simulink model "ACC_FFNN_trainlm_10_10_10_Nor_Sat_Feb_15_RepFast"  (R2021a)
settings: Solver=FixedStepAuto  StartTime=0.0  StopTime=T  RelTol=1e-3
InitFcn:
  | seed = randi(10000);
StartFcn:
  | seed = randi(10000);
undefined symbols (not defined in the file): amax_ego, amin_ego, patch_sig, safe_patch_sig, sw, t_gap, Ts, v0_ego, v0_lead, v_set, x0_ego, x0_lead, x_gain, x_offset, y_gain, y_offset
libraries: neural x35, simulink x3
(part 1 of 2)
settings Model: SimulationMode=accelerator  Creator=The MathWorks, Inc.  LastModifiedBy=deyun
settings SolverCC: AlgebraicLoopSolver=TrustRegion
settings DataIOCC: ReturnWorkspaceOutputs=off
settings DebuggingCC: ArithmeticOperatorsInVariantConditions=warning
settings SFSimCC: SimUseLocalCustomCode=off  CustomCodeUndefinedFunction=UseInterfaceOnly
settings RTWCC: RTWUseLocalCustomCode=off
settings CodeAppCC: StateflowObjectComments=on
settings ConfigComp: CovBoundaryAbsTol=1.0e-5

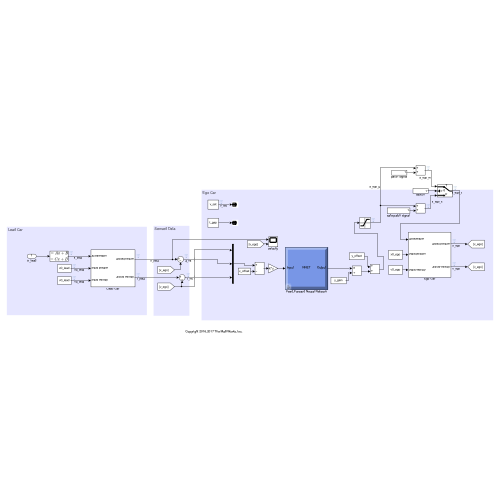
[thumbnail: Simulink's stored preview of the top-level diagram]
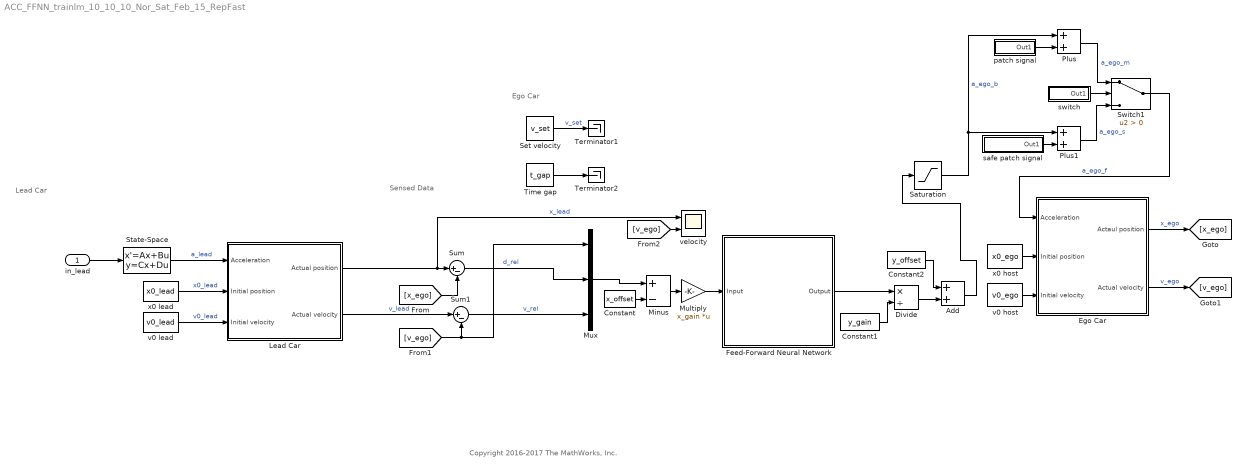
== system ACC_FFNN_trainlm_10_10_10_Nor_Sat_Feb_15_RepFast ==
  note: Sensed Data
  note: Lead Car
  note: Ego Car
  note: Copyright 2016-2017 The MathWorks, Inc.
  in_lead : Inport
  Add : Sum
  Constant : Constant  Value=x_offset
  Constant1 : Constant  Value=y_gain
  Constant2 : Constant  Value=y_offset
  Divide : Product  Inputs=*/
  Ego Car : Subsystem
  Feed-Forward Neural Network : Subsystem
      mask help: Feed-Forward Neural Network
      mask Display: e = 0.06;c1 = [120 150 230]/255;c2 = ([120 150 230]+0)/383;c3 = ([120 150 230]+128)/383;patch([0 1 1 0],[0 0 1 1],c1);patch([0 1 1 1-e 1-e 0+e],[0 0 1 1-e 0+e 0+e],c2);patch([0 0 1 1-e 0+e 0+e],[0 1 1 1-e 1-e 0+e],c3);plot([0 1 1 0 0],[0 0 1 1 0]);fprintf('NNET');port_label('input',1,' Input');port_label('output',1,'Output ');
  Lead Car : Subsystem
  Minus : Sum  Inputs=+-
  Multiply : Gain  Gain=x_gain  Multiplication=Matrix(K*u)
  Mux : Mux  Inputs=3
  Plus : Sum
  Plus1 : Sum
  Saturation : Saturate  UpperLimit=amax_ego  LowerLimit=amin_ego
  Set velocity : Constant  Value=v_set  SampleTime=Ts
  State-Space : StateSpace  A=-10  B=10  D=0  InitialCondition=0
  Sum : Sum  Inputs=|+-
  Sum1 : Sum  Inputs=|+-
  Switch1 : Switch  Criteria=u2 > Threshold
  Terminator1 : Terminator
  Terminator2 : Terminator
  Time gap : Constant  Value=t_gap  SampleTime=Ts
  patch signal : Subsystem
  safe patch signal : Subsystem
  switch : Subsystem
  v0 host : Constant  Value=v0_ego  SampleTime=Ts
  v0 lead : Constant  Value=v0_lead  SampleTime=Ts
  velocity : Scope  NumInputPorts=2
  x0 host : Constant  Value=x0_ego  SampleTime=Ts
  x0 lead : Constant  Value=x0_lead  SampleTime=Ts
  wires:
  x0 lead/1 -> Lead Car/2(Initial position)  "x0_lead"
  v0 lead/1 -> Lead Car/3(Initial velocity)  "v0_lead"
  x0 host/1 -> Ego Car/2(Initial position)
  v0 host/1 -> Ego Car/3(Initial velocity)
  Feed-Forward Neural Network/1(Output) -> Divide/1
  Lead Car/1(Actual position) -> velocity/1, Sum/1  "x_lead"
  Sum1/1 -> Mux/3  "v_rel"
  State-Space/1 -> Lead Car/1(Acceleration)  "a_lead"
  Lead Car/2(Actual velocity) -> Sum1/1  "v_lead"
  in_lead/1 -> State-Space/1
  Mux/1 -> Minus/1
  Add/1 -> Saturation/1
  Multiply/1 -> Feed-Forward Neural Network/1(Input)
  Set velocity/1 -> Terminator1/1  "v_set"
  Time gap/1 -> Terminator2/1
  Constant/1 -> Minus/2
  Minus/1 -> Multiply/1
  Constant1/1 -> Divide/2
  Divide/1 -> Add/2
  Constant2/1 -> Add/1
  Ego Car/1(Actaul position) -> [x_ego]  "x_ego"
  [x_ego] -> Sum/2
  Ego Car/2(Actual velocity) -> [v_ego]  "v_ego"
  [v_ego] -> Mux/1, Sum1/2
  [v_ego] -> velocity/2
  Sum/1 -> Mux/2  "d_rel"
  Saturation/1 -> Plus/1, Plus1/1  "a_ego_b"
  Plus1/1 -> Switch1/3  "a_ego_s"
  Switch1/1 -> Ego Car/1(Acceleration)  "a_ego_f"
  Plus/1 -> Switch1/1  "a_ego_m"
  patch signal/1(Out1) -> Plus/2
  safe patch signal/1(Out1) -> Plus1/2
  switch/1(Out1) -> Switch1/2

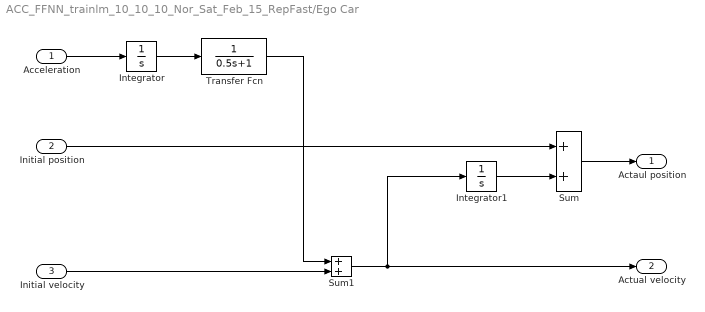
== system ACC_FFNN_trainlm_10_10_10_Nor_Sat_Feb_15_RepFast/Ego Car ==
  Acceleration : Inport
  Initial position : Inport  Port=2
  Initial velocity : Inport  Port=3
  Integrator : Integrator
  Integrator1 : Integrator
  Sum : Sum
  Sum1 : Sum
  Transfer Fcn : TransferFcn  Denominator=[0.5 1]
  Actaul position : Outport  VectorParamsAs1DForOutWhenUnconnected=off
  Actual velocity : Outport  Port=2  VectorParamsAs1DForOutWhenUnconnected=off
  wires:
  Sum1/1 -> Integrator1/1, Actual velocity/1
  Initial velocity/1 -> Sum1/2
  Sum/1 -> Actaul position/1
  Transfer Fcn/1 -> Sum1/1
  Integrator/1 -> Transfer Fcn/1
  Acceleration/1 -> Integrator/1
  Initial position/1 -> Sum/1
  Integrator1/1 -> Sum/2

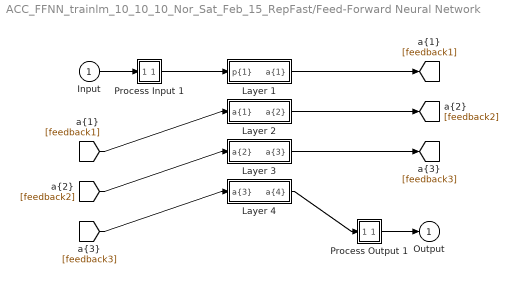
== system ACC_FFNN_trainlm_10_10_10_Nor_Sat_Feb_15_RepFast/Feed-Forward Neural Network ==
  Input : Inport  PortDimensions=3
      mask Display: e = 0.06;c1 = [120 230 180]/255;c2 = ([120 230 180]+0)/(256+128);c3 = ([120 230 180]+128)/(256+128);patch([0 1 1 0],[0 0 1 1],c1);patch([0 1 1 1-e 1-e 0+e],[0 0 1 1-e 0+e 0+e],c2);patch([0 0 1 1-e 0+e 0+e],[0 1 1 1-e 1-e 0+e],c3);plot([0 1 1 0 0],[0 0 1 1 0]);
  Layer 1 : Subsystem
      mask Display: e = 0.06;c1 = [120 150 230]/255;c2 = ([120 150 230]+0)/383;c3 = ([120 150 230]+128)/383;patch([0 1 1 0],[0 0 1 1],c1);patch([0 1 1 1-e 1-e 0+e],[0 0 1 1-e 0+e 0+e],c2);patch([0 0 1 1-e 0+e 0+e],[0 1 1 1-e 1-e 0+e],c3);plot([0 1 1 0 0],[0 0 1 1 0]);
  Layer 2 : Subsystem
      mask Display: e = 0.06;c1 = [120 150 230]/255;c2 = ([120 150 230]+0)/383;c3 = ([120 150 230]+128)/383;patch([0 1 1 0],[0 0 1 1],c1);patch([0 1 1 1-e 1-e 0+e],[0 0 1 1-e 0+e 0+e],c2);patch([0 0 1 1-e 0+e 0+e],[0 1 1 1-e 1-e 0+e],c3);plot([0 1 1 0 0],[0 0 1 1 0]);
  Layer 3 : Subsystem
      mask Display: e = 0.06;c1 = [120 150 230]/255;c2 = ([120 150 230]+0)/383;c3 = ([120 150 230]+128)/383;patch([0 1 1 0],[0 0 1 1],c1);patch([0 1 1 1-e 1-e 0+e],[0 0 1 1-e 0+e 0+e],c2);patch([0 0 1 1-e 0+e 0+e],[0 1 1 1-e 1-e 0+e],c3);plot([0 1 1 0 0],[0 0 1 1 0]);
  Layer 4 : Subsystem
      mask Display: e = 0.06;c1 = [120 150 230]/255;c2 = ([120 150 230]+0)/383;c3 = ([120 150 230]+128)/383;patch([0 1 1 0],[0 0 1 1],c1);patch([0 1 1 1-e 1-e 0+e],[0 0 1 1-e 0+e 0+e],c2);patch([0 0 1 1-e 0+e 0+e],[0 1 1 1-e 1-e 0+e],c3);plot([0 1 1 0 0],[0 0 1 1 0]);
  Process Input 1 : Subsystem
      mask Display: e = 0.06;c1 = [120 150 230]/255;c2 = ([120 150 230]+0)/383;c3 = ([120 150 230]+128)/383;patch([0 1 1 0],[0 0 1 1],c1);patch([0 1 1 1-e 1-e 0+e],[0 0 1 1-e 0+e 0+e],c2);patch([0 0 1 1-e 0+e 0+e],[0 1 1 1-e 1-e 0+e],c3);plot([0 1 1 0 0],[0 0 1 1 0]);
  Process Output 1 : Subsystem
      mask Display: e = 0.06;c1 = [120 150 230]/255;c2 = ([120 150 230]+0)/383;c3 = ([120 150 230]+128)/383;patch([0 1 1 0],[0 0 1 1],c1);patch([0 1 1 1-e 1-e 0+e],[0 0 1 1-e 0+e 0+e],c2);patch([0 0 1 1-e 0+e 0+e],[0 1 1 1-e 1-e 0+e],c3);plot([0 1 1 0 0],[0 0 1 1 0]);
  Output : Outport  InitialOutput=0
      mask Display: e = 0.06;c1 = [120 230 180]/255;c2 = ([120 230 180]+0)/(256+128);c3 = ([120 230 180]+128)/(256+128);patch([0 1 1 0],[0 0 1 1],c1);patch([0 1 1 1-e 1-e 0+e],[0 0 1 1-e 0+e 0+e],c2);patch([0 0 1 1-e 0+e 0+e],[0 1 1 1-e 1-e 0+e],c3);plot([0 1 1 0 0],[0 0 1 1 0]);
  wires:
  Input/1 -> Process Input 1/1(x)
  Process Output 1/1(y) -> Output/1
  Process Input 1/1(p) -> Layer 1/1("p{1}")
  Layer 1/1("a{1}") -> [feedback1]
  [feedback1] -> Layer 2/1("a{1} ")
  Layer 2/1("a{2}") -> [feedback2]
  [feedback2] -> Layer 3/1("a{2} ")
  Layer 3/1("a{3}") -> [feedback3]
  [feedback3] -> Layer 4/1("a{3} ")
  Layer 4/1("a{4}") -> Process Output 1/1(a)

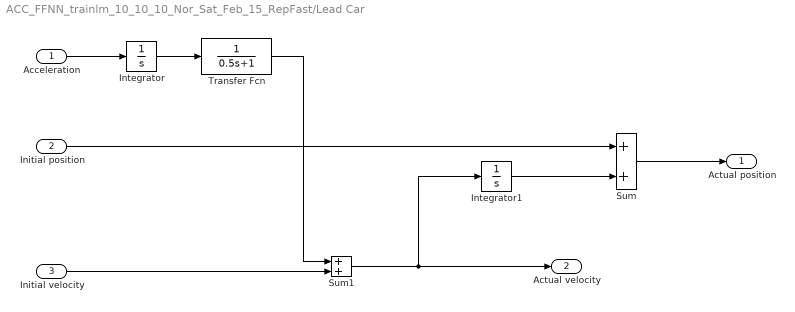
== system ACC_FFNN_trainlm_10_10_10_Nor_Sat_Feb_15_RepFast/Lead Car ==
  Acceleration : Inport
  Initial position : Inport  Port=2
  Initial velocity : Inport  Port=3
  Integrator : Integrator
  Integrator1 : Integrator
  Sum : Sum
  Sum1 : Sum
  Transfer Fcn : TransferFcn  Denominator=[0.5 1]
  Actual position : Outport  VectorParamsAs1DForOutWhenUnconnected=off
  Actual velocity : Outport  Port=2  VectorParamsAs1DForOutWhenUnconnected=off
  wires:
  Transfer Fcn/1 -> Sum1/1
  Initial velocity/1 -> Sum1/2
  Sum/1 -> Actual position/1
  Integrator/1 -> Transfer Fcn/1
  Sum1/1 -> Integrator1/1, Actual velocity/1
  Acceleration/1 -> Integrator/1
  Initial position/1 -> Sum/1
  Integrator1/1 -> Sum/2

== system ACC_FFNN_trainlm_10_10_10_Nor_Sat_Feb_15_RepFast/patch signal ==
  Sample index : simulink/Sources/Counter Limited  uplimit=numel(patch_sig)-1  tsamp=Ts
  Sample value : LookupNDDirect  NumberOfTableDimensions=1  Table=patch_sig  DiagnosticForOutOfRangeInput=None
  Out1 : Outport
  wires:
  Sample index/1 -> Sample value/1
  Sample value/1 -> Out1/1

== system ACC_FFNN_trainlm_10_10_10_Nor_Sat_Feb_15_RepFast/safe patch signal ==
  Sample index : simulink/Sources/Counter Limited  uplimit=numel(safe_patch_sig)-1  tsamp=Ts
  Sample value : LookupNDDirect  NumberOfTableDimensions=1  Table=safe_patch_sig  DiagnosticForOutOfRangeInput=None
  Out1 : Outport
  wires:
  Sample index/1 -> Sample value/1
  Sample value/1 -> Out1/1

== system ACC_FFNN_trainlm_10_10_10_Nor_Sat_Feb_15_RepFast/switch ==
  Sample index : simulink/Sources/Counter Limited  uplimit=numel(sw)-1  tsamp=Ts
  Sample value : LookupNDDirect  NumberOfTableDimensions=1  Table=sw  DiagnosticForOutOfRangeInput=None
  Out1 : Outport
  wires:
  Sample index/1 -> Sample value/1
  Sample value/1 -> Out1/1

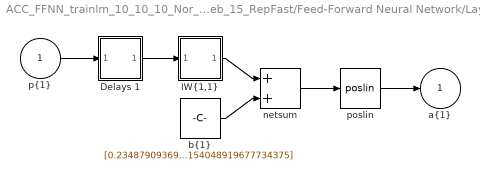
== system ACC_FFNN_trainlm_10_10_10_Nor_Sat_Feb_15_RepFast/Feed-Forward Neural Network/Layer 1 ==
  "p{1}" : Inport  PortDimensions=3
      mask Display: e = 0.06;c1 = [120 230 180]/255;c2 = ([120 230 180]+0)/(256+128);c3 = ([120 230 180]+128)/(256+128);patch([0 1 1 0],[0 0 1 1],c1);patch([0 1 1 1-e 1-e 0+e],[0 0 1 1-e 0+e 0+e],c2);patch([0 0 1 1-e 0+e 0+e],[0 1 1 1-e 1-e 0+e],c3);plot([0 1 1 0 0],[0 0 1 1 0]);
  Delays 1 : Subsystem
      mask Display: e = 0.06;c1 = [120 150 230]/255;c2 = ([120 150 230]+0)/383;c3 = ([120 150 230]+128)/383;patch([0 1 1 0],[0 0 1 1],c1);patch([0 1 1 1-e 1-e 0+e],[0 0 1 1-e 0+e 0+e],c2);patch([0 0 1 1-e 0+e 0+e],[0 1 1 1-e 1-e 0+e],c3);plot([0 1 1 0 0],[0 0 1 1 0]);disp('0');
  "IW{1,1}" : Subsystem
      mask Display: e = 0.06;c1 = [120 150 230]/255;c2 = ([120 150 230]+0)/383;c3 = ([120 150 230]+128)/383;patch([0 1 1 0],[0 0 1 1],c1);patch([0 1 1 1-e 1-e 0+e],[0 0 1 1-e 0+e 0+e],c2);patch([0 0 1 1-e 0+e 0+e],[0 1 1 1-e 1-e 0+e],c3);plot([0 1 1 0 0],[0 0 1 1 0]);disp('W');
  "b{1}" : Constant  Value=[0.2348790936912676652337239602275076322257518768310546875;-0.47557650443830912223575069219805300235748291015625;0.78952949301104913271132090812898240983486175537109375;0.27963461410623235980921208465588279068470001220703125;-0.65288334165578765233561853165156207978725433349609375;-0.6252719481796160660991290569654665887355804443359375;-0.285681783449709458810872320100315846502780914306640625;-0.362443396148235397191683659912087023258209228515625;-0.169633536236455551016177878409507684409618377685546875;0.07730292547507398859263361146076931618154048919677734375]
      mask Display: e = 0.06;c1 = [120 150 230]/255;c2 = ([120 150 230]+0)/383;c3 = ([120 150 230]+128)/383;patch([0 1 1 0],[0 0 1 1],c1);patch([0 1 1 1-e 1-e 0+e],[0 0 1 1-e 0+e 0+e],c2);patch([0 0 1 1-e 0+e 0+e],[0 1 1 1-e 1-e 0+e],c3);plot([0 1 1 0 0],[0 0 1 1 0]);disp('b');
  netsum : Sum  Inputs=2  InputSameDT=on  SaturateOnIntegerOverflow=on  OutDataTypeStr=Inherit: Same as first input
      mask Display: e = 0.06;c1 = [120 150 230]/255;c2 = ([120 150 230]+0)/383;c3 = ([120 150 230]+128)/383;patch([0 1 1 0],[0 0 1 1],c1);patch([0 1 1 1-e 1-e 0+e],[0 0 1 1-e 0+e 0+e],c2);patch([0 0 1 1-e 0+e 0+e],[0 1 1 1-e 1-e 0+e],c3);plot([0 1 1 0 0],[0 0 1 1 0]);disp('+');
  poslin : neural/Transfer Functions/poslin
  "a{1}" : Outport  InitialOutput=[0;0;0;0;0;0;0;0;0;0]
      mask Display: e = 0.06;c1 = [120 230 180]/255;c2 = ([120 230 180]+0)/(256+128);c3 = ([120 230 180]+128)/(256+128);patch([0 1 1 0],[0 0 1 1],c1);patch([0 1 1 1-e 1-e 0+e],[0 0 1 1-e 0+e 0+e],c2);patch([0 0 1 1-e 0+e 0+e],[0 1 1 1-e 1-e 0+e],c3);plot([0 1 1 0 0],[0 0 1 1 0]);
  wires:
  "p{1}"/1 -> Delays 1/1("p{1}")
  Delays 1/1("pd{1,1}") -> "IW{1,1}"/1("pd{1,1}")
  "IW{1,1}"/1("iz{1,1}") -> netsum/1
  "b{1}"/1 -> netsum/2
  netsum/1 -> poslin/1
  poslin/1 -> "a{1}"/1

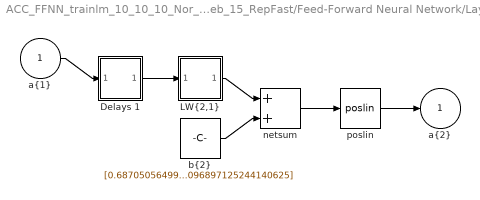
== system ACC_FFNN_trainlm_10_10_10_Nor_Sat_Feb_15_RepFast/Feed-Forward Neural Network/Layer 2 ==
  "a{1} " : Inport  PortDimensions=10
      mask Display: e = 0.06;c1 = [120 230 180]/255;c2 = ([120 230 180]+0)/(256+128);c3 = ([120 230 180]+128)/(256+128);patch([0 1 1 0],[0 0 1 1],c1);patch([0 1 1 1-e 1-e 0+e],[0 0 1 1-e 0+e 0+e],c2);patch([0 0 1 1-e 0+e 0+e],[0 1 1 1-e 1-e 0+e],c3);plot([0 1 1 0 0],[0 0 1 1 0]);
  Delays 1 : Subsystem
      mask Display: e = 0.06;c1 = [120 150 230]/255;c2 = ([120 150 230]+0)/383;c3 = ([120 150 230]+128)/383;patch([0 1 1 0],[0 0 1 1],c1);patch([0 1 1 1-e 1-e 0+e],[0 0 1 1-e 0+e 0+e],c2);patch([0 0 1 1-e 0+e 0+e],[0 1 1 1-e 1-e 0+e],c3);plot([0 1 1 0 0],[0 0 1 1 0]);disp('0');
  "LW{2,1}" : Subsystem
      mask Display: e = 0.06;c1 = [120 150 230]/255;c2 = ([120 150 230]+0)/383;c3 = ([120 150 230]+128)/383;patch([0 1 1 0],[0 0 1 1],c1);patch([0 1 1 1-e 1-e 0+e],[0 0 1 1-e 0+e 0+e],c2);patch([0 0 1 1-e 0+e 0+e],[0 1 1 1-e 1-e 0+e],c3);plot([0 1 1 0 0],[0 0 1 1 0]);disp('W');
  "b{2}" : Constant  Value=[0.68705056499902916744559888684307225048542022705078125;0.94653343063350003916411878890357911586761474609375;-0.94981534008346379938103609674726612865924835205078125;0.43723562506075897005075603374280035495758056640625;-0.46176114720288818915605588699690997600555419921875;-0.360550158804355092012627892472664825618267059326171875;-0.214341347450948627173517024857574142515659332275390625;1.1655184078745570719348734201048500835895538330078125;-0.1645117913666755971036081973579712212085723876953125;1.350983412230919444851906519033946096897125244140625]
      mask Display: e = 0.06;c1 = [120 150 230]/255;c2 = ([120 150 230]+0)/383;c3 = ([120 150 230]+128)/383;patch([0 1 1 0],[0 0 1 1],c1);patch([0 1 1 1-e 1-e 0+e],[0 0 1 1-e 0+e 0+e],c2);patch([0 0 1 1-e 0+e 0+e],[0 1 1 1-e 1-e 0+e],c3);plot([0 1 1 0 0],[0 0 1 1 0]);disp('b');
  netsum : Sum  Inputs=2  InputSameDT=on  SaturateOnIntegerOverflow=on  OutDataTypeStr=Inherit: Same as first input
      mask Display: e = 0.06;c1 = [120 150 230]/255;c2 = ([120 150 230]+0)/383;c3 = ([120 150 230]+128)/383;patch([0 1 1 0],[0 0 1 1],c1);patch([0 1 1 1-e 1-e 0+e],[0 0 1 1-e 0+e 0+e],c2);patch([0 0 1 1-e 0+e 0+e],[0 1 1 1-e 1-e 0+e],c3);plot([0 1 1 0 0],[0 0 1 1 0]);disp('+');
  poslin : neural/Transfer Functions/poslin
  "a{2}" : Outport  InitialOutput=[0;0;0;0;0;0;0;0;0;0]
      mask Display: e = 0.06;c1 = [120 230 180]/255;c2 = ([120 230 180]+0)/(256+128);c3 = ([120 230 180]+128)/(256+128);patch([0 1 1 0],[0 0 1 1],c1);patch([0 1 1 1-e 1-e 0+e],[0 0 1 1-e 0+e 0+e],c2);patch([0 0 1 1-e 0+e 0+e],[0 1 1 1-e 1-e 0+e],c3);plot([0 1 1 0 0],[0 0 1 1 0]);
  wires:
  "a{1} "/1 -> Delays 1/1("p{2}")
  Delays 1/1("pd{2,1}") -> "LW{2,1}"/1("ad{2,1}")
  "LW{2,1}"/1("lz{2,1}") -> netsum/1
  "b{2}"/1 -> netsum/2
  netsum/1 -> poslin/1
  poslin/1 -> "a{2}"/1

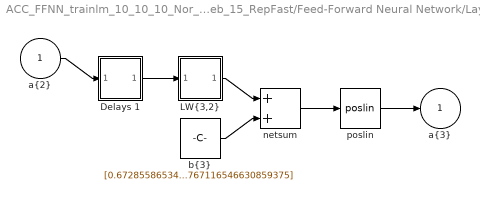
== system ACC_FFNN_trainlm_10_10_10_Nor_Sat_Feb_15_RepFast/Feed-Forward Neural Network/Layer 3 ==
  "a{2} " : Inport  PortDimensions=10
      mask Display: e = 0.06;c1 = [120 230 180]/255;c2 = ([120 230 180]+0)/(256+128);c3 = ([120 230 180]+128)/(256+128);patch([0 1 1 0],[0 0 1 1],c1);patch([0 1 1 1-e 1-e 0+e],[0 0 1 1-e 0+e 0+e],c2);patch([0 0 1 1-e 0+e 0+e],[0 1 1 1-e 1-e 0+e],c3);plot([0 1 1 0 0],[0 0 1 1 0]);
  Delays 1 : Subsystem
      mask Display: e = 0.06;c1 = [120 150 230]/255;c2 = ([120 150 230]+0)/383;c3 = ([120 150 230]+128)/383;patch([0 1 1 0],[0 0 1 1],c1);patch([0 1 1 1-e 1-e 0+e],[0 0 1 1-e 0+e 0+e],c2);patch([0 0 1 1-e 0+e 0+e],[0 1 1 1-e 1-e 0+e],c3);plot([0 1 1 0 0],[0 0 1 1 0]);disp('0');
  "LW{3,2}" : Subsystem
      mask Display: e = 0.06;c1 = [120 150 230]/255;c2 = ([120 150 230]+0)/383;c3 = ([120 150 230]+128)/383;patch([0 1 1 0],[0 0 1 1],c1);patch([0 1 1 1-e 1-e 0+e],[0 0 1 1-e 0+e 0+e],c2);patch([0 0 1 1-e 0+e 0+e],[0 1 1 1-e 1-e 0+e],c3);plot([0 1 1 0 0],[0 0 1 1 0]);disp('W');
  "b{3}" : Constant  Value=[0.6728558653448353243931023826007731258869171142578125;-0.9976978857417855284239749380503781139850616455078125;-0.3335507224139184767608412585104815661907196044921875;-0.1880800197195158507401657743685063906013965606689453125;-0.0781672679420719607179535159957595169544219970703125;0.54021632205061675957580291651538573205471038818359375;-0.50845547786183120653191735982545651495456695556640625;0.56201675169722253855297822155989706516265869140625;-0.057285692578776803429718711413443088531494140625;-0.96286216425843418331709244739613495767116546630859375]
      mask Display: e = 0.06;c1 = [120 150 230]/255;c2 = ([120 150 230]+0)/383;c3 = ([120 150 230]+128)/383;patch([0 1 1 0],[0 0 1 1],c1);patch([0 1 1 1-e 1-e 0+e],[0 0 1 1-e 0+e 0+e],c2);patch([0 0 1 1-e 0+e 0+e],[0 1 1 1-e 1-e 0+e],c3);plot([0 1 1 0 0],[0 0 1 1 0]);disp('b');
  netsum : Sum  Inputs=2  InputSameDT=on  SaturateOnIntegerOverflow=on  OutDataTypeStr=Inherit: Same as first input
      mask Display: e = 0.06;c1 = [120 150 230]/255;c2 = ([120 150 230]+0)/383;c3 = ([120 150 230]+128)/383;patch([0 1 1 0],[0 0 1 1],c1);patch([0 1 1 1-e 1-e 0+e],[0 0 1 1-e 0+e 0+e],c2);patch([0 0 1 1-e 0+e 0+e],[0 1 1 1-e 1-e 0+e],c3);plot([0 1 1 0 0],[0 0 1 1 0]);disp('+');
  poslin : neural/Transfer Functions/poslin
  "a{3}" : Outport  InitialOutput=[0;0;0;0;0;0;0;0;0;0]
      mask Display: e = 0.06;c1 = [120 230 180]/255;c2 = ([120 230 180]+0)/(256+128);c3 = ([120 230 180]+128)/(256+128);patch([0 1 1 0],[0 0 1 1],c1);patch([0 1 1 1-e 1-e 0+e],[0 0 1 1-e 0+e 0+e],c2);patch([0 0 1 1-e 0+e 0+e],[0 1 1 1-e 1-e 0+e],c3);plot([0 1 1 0 0],[0 0 1 1 0]);
  wires:
  "a{2} "/1 -> Delays 1/1("p{3}")
  Delays 1/1("pd{3,2}") -> "LW{3,2}"/1("ad{3,2}")
  "LW{3,2}"/1("lz{3,2}") -> netsum/1
  "b{3}"/1 -> netsum/2
  netsum/1 -> poslin/1
  poslin/1 -> "a{3}"/1

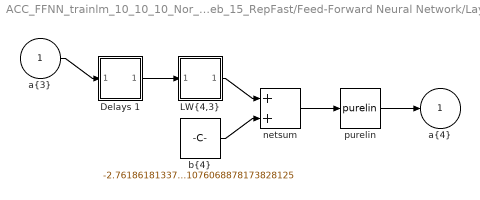
== system ACC_FFNN_trainlm_10_10_10_Nor_Sat_Feb_15_RepFast/Feed-Forward Neural Network/Layer 4 ==
  "a{3} " : Inport  PortDimensions=10
      mask Display: e = 0.06;c1 = [120 230 180]/255;c2 = ([120 230 180]+0)/(256+128);c3 = ([120 230 180]+128)/(256+128);patch([0 1 1 0],[0 0 1 1],c1);patch([0 1 1 1-e 1-e 0+e],[0 0 1 1-e 0+e 0+e],c2);patch([0 0 1 1-e 0+e 0+e],[0 1 1 1-e 1-e 0+e],c3);plot([0 1 1 0 0],[0 0 1 1 0]);
  Delays 1 : Subsystem
      mask Display: e = 0.06;c1 = [120 150 230]/255;c2 = ([120 150 230]+0)/383;c3 = ([120 150 230]+128)/383;patch([0 1 1 0],[0 0 1 1],c1);patch([0 1 1 1-e 1-e 0+e],[0 0 1 1-e 0+e 0+e],c2);patch([0 0 1 1-e 0+e 0+e],[0 1 1 1-e 1-e 0+e],c3);plot([0 1 1 0 0],[0 0 1 1 0]);disp('0');
  "LW{4,3}" : Subsystem
      mask Display: e = 0.06;c1 = [120 150 230]/255;c2 = ([120 150 230]+0)/383;c3 = ([120 150 230]+128)/383;patch([0 1 1 0],[0 0 1 1],c1);patch([0 1 1 1-e 1-e 0+e],[0 0 1 1-e 0+e 0+e],c2);patch([0 0 1 1-e 0+e 0+e],[0 1 1 1-e 1-e 0+e],c3);plot([0 1 1 0 0],[0 0 1 1 0]);disp('W');
  "b{4}" : Constant  Value=-2.7618618133792427471462360699661076068878173828125
      mask Display: e = 0.06;c1 = [120 150 230]/255;c2 = ([120 150 230]+0)/383;c3 = ([120 150 230]+128)/383;patch([0 1 1 0],[0 0 1 1],c1);patch([0 1 1 1-e 1-e 0+e],[0 0 1 1-e 0+e 0+e],c2);patch([0 0 1 1-e 0+e 0+e],[0 1 1 1-e 1-e 0+e],c3);plot([0 1 1 0 0],[0 0 1 1 0]);disp('b');
  netsum : Sum  Inputs=2  InputSameDT=on  SaturateOnIntegerOverflow=on  OutDataTypeStr=Inherit: Same as first input
      mask Display: e = 0.06;c1 = [120 150 230]/255;c2 = ([120 150 230]+0)/383;c3 = ([120 150 230]+128)/383;patch([0 1 1 0],[0 0 1 1],c1);patch([0 1 1 1-e 1-e 0+e],[0 0 1 1-e 0+e 0+e],c2);patch([0 0 1 1-e 0+e 0+e],[0 1 1 1-e 1-e 0+e],c3);plot([0 1 1 0 0],[0 0 1 1 0]);disp('+');
  purelin : neural/Transfer Functions/purelin
  "a{4}" : Outport  InitialOutput=0
      mask Display: e = 0.06;c1 = [120 230 180]/255;c2 = ([120 230 180]+0)/(256+128);c3 = ([120 230 180]+128)/(256+128);patch([0 1 1 0],[0 0 1 1],c1);patch([0 1 1 1-e 1-e 0+e],[0 0 1 1-e 0+e 0+e],c2);patch([0 0 1 1-e 0+e 0+e],[0 1 1 1-e 1-e 0+e],c3);plot([0 1 1 0 0],[0 0 1 1 0]);
  wires:
  "a{3} "/1 -> Delays 1/1("p{4}")
  Delays 1/1("pd{4,3}") -> "LW{4,3}"/1("ad{4,3}")
  "LW{4,3}"/1("lz{4,3}") -> netsum/1
  "b{4}"/1 -> netsum/2
  netsum/1 -> purelin/1
  purelin/1 -> "a{4}"/1

== system ACC_FFNN_trainlm_10_10_10_Nor_Sat_Feb_15_RepFast/Feed-Forward Neural Network/Process Input 1 ==
  x : Inport  PortDimensions=3
      mask Display: e = 0.06;c1 = [120 230 180]/255;c2 = ([120 230 180]+0)/(256+128);c3 = ([120 230 180]+128)/(256+128);patch([0 1 1 0],[0 0 1 1],c1);patch([0 1 1 1-e 1-e 0+e],[0 0 1 1-e 0+e 0+e],c2);patch([0 0 1 1-e 0+e 0+e],[0 1 1 1-e 1-e 0+e],c3);plot([0 1 1 0 0],[0 0 1 1 0]);
  p : Outport  PortDimensions=3
      mask Display: e = 0.06;c1 = [120 230 180]/255;c2 = ([120 230 180]+0)/(256+128);c3 = ([120 230 180]+128)/(256+128);patch([0 1 1 0],[0 0 1 1],c1);patch([0 1 1 1-e 1-e 0+e],[0 0 1 1-e 0+e 0+e],c2);patch([0 0 1 1-e 0+e 0+e],[0 1 1 1-e 1-e 0+e],c3);plot([0 1 1 0 0],[0 0 1 1 0]);
  wires:
  x/1 -> p/1

== system ACC_FFNN_trainlm_10_10_10_Nor_Sat_Feb_15_RepFast/Feed-Forward Neural Network/Process Output 1 ==
  a : Inport  PortDimensions=1
      mask Display: e = 0.06;c1 = [120 230 180]/255;c2 = ([120 230 180]+0)/(256+128);c3 = ([120 230 180]+128)/(256+128);patch([0 1 1 0],[0 0 1 1],c1);patch([0 1 1 1-e 1-e 0+e],[0 0 1 1-e 0+e 0+e],c2);patch([0 0 1 1-e 0+e 0+e],[0 1 1 1-e 1-e 0+e],c3);plot([0 1 1 0 0],[0 0 1 1 0]);
  y : Outport  PortDimensions=1
      mask Display: e = 0.06;c1 = [120 230 180]/255;c2 = ([120 230 180]+0)/(256+128);c3 = ([120 230 180]+128)/(256+128);patch([0 1 1 0],[0 0 1 1],c1);patch([0 1 1 1-e 1-e 0+e],[0 0 1 1-e 0+e 0+e],c2);patch([0 0 1 1-e 0+e 0+e],[0 1 1 1-e 1-e 0+e],c3);plot([0 1 1 0 0],[0 0 1 1 0]);
  wires:
  a/1 -> y/1

== system ACC_FFNN_trainlm_10_10_10_Nor_Sat_Feb_15_RepFast/Feed-Forward Neural Network/Layer 1/Delays 1 ==
  "p{1}" : Inport  PortDimensions=3
      mask Display: e = 0.06;c1 = [120 230 180]/255;c2 = ([120 230 180]+0)/(256+128);c3 = ([120 230 180]+128)/(256+128);patch([0 1 1 0],[0 0 1 1],c1);patch([0 1 1 1-e 1-e 0+e],[0 0 1 1-e 0+e 0+e],c2);patch([0 0 1 1-e 0+e 0+e],[0 1 1 1-e 1-e 0+e],c3);plot([0 1 1 0 0],[0 0 1 1 0]);
  mux : Mux  Inputs=1
      mask Display: e = 0.06;c1 = [120 150 230]/255;c2 = ([120 150 230]+0)/383;c3 = ([120 150 230]+128)/383;patch([0 1 1 0],[0 0 1 1],c1);patch([0 1 1 1-e 1-e 0+e],[0 0 1 1-e 0+e 0+e],c2);patch([0 0 1 1-e 0+e 0+e],[0 1 1 1-e 1-e 0+e],c3);plot([0 1 1 0 0],[0 0 1 1 0]);disp('Mux')
  "pd{1,1}" : Outport
      mask Display: e = 0.06;c1 = [120 230 180]/255;c2 = ([120 230 180]+0)/(256+128);c3 = ([120 230 180]+128)/(256+128);patch([0 1 1 0],[0 0 1 1],c1);patch([0 1 1 1-e 1-e 0+e],[0 0 1 1-e 0+e 0+e],c2);patch([0 0 1 1-e 0+e 0+e],[0 1 1 1-e 1-e 0+e],c3);plot([0 1 1 0 0],[0 0 1 1 0]);
  wires:
  "p{1}"/1 -> mux/1
  mux/1 -> "pd{1,1}"/1

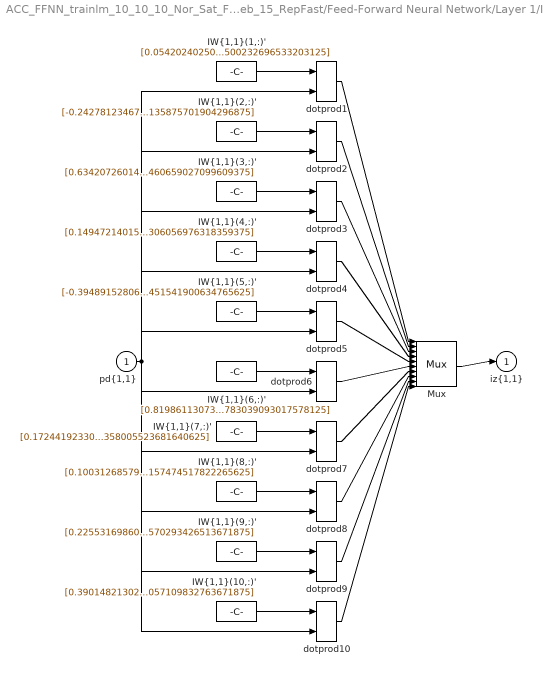
== system ACC_FFNN_trainlm_10_10_10_Nor_Sat_Feb_15_RepFast/Feed-Forward Neural Network/Layer 1/IW{1,1} ==
  "pd{1,1}" : Inport  PortDimensions=3
      mask Display: e = 0.06;c1 = [120 230 180]/255;c2 = ([120 230 180]+0)/(256+128);c3 = ([120 230 180]+128)/(256+128);patch([0 1 1 0],[0 0 1 1],c1);patch([0 1 1 1-e 1-e 0+e],[0 0 1 1-e 0+e 0+e],c2);patch([0 0 1 1-e 0+e 0+e],[0 1 1 1-e 1-e 0+e],c3);plot([0 1 1 0 0],[0 0 1 1 0]);
  "IW{1,1}(1,:)'" : Constant  Value=[0.054202402501876877083386574440737604163587093353271484375;1.282306499887972517370826608384959399700164794921875;-0.447846071912107124290969295543618500232696533203125]
      mask Display: e = 0.06;c1 = [120 150 230]/255;c2 = ([120 150 230]+0)/383;c3 = ([120 150 230]+128)/383;patch([0 1 1 0],[0 0 1 1],c1);patch([0 1 1 1-e 1-e 0+e],[0 0 1 1-e 0+e 0+e],c2);patch([0 0 1 1-e 0+e 0+e],[0 1 1 1-e 1-e 0+e],c3);plot([0 1 1 0 0],[0 0 1 1 0]);disp('Weights');
  "IW{1,1}(10,:)'" : Constant  Value=[0.3901482130268687509300207238993607461452484130859375;-4.59823632446252172911727029713802039623260498046875;-0.6222373009711190672277325575123541057109832763671875]
      mask Display: e = 0.06;c1 = [120 150 230]/255;c2 = ([120 150 230]+0)/383;c3 = ([120 150 230]+128)/383;patch([0 1 1 0],[0 0 1 1],c1);patch([0 1 1 1-e 1-e 0+e],[0 0 1 1-e 0+e 0+e],c2);patch([0 0 1 1-e 0+e 0+e],[0 1 1 1-e 1-e 0+e],c3);plot([0 1 1 0 0],[0 0 1 1 0]);disp('Weights');
  "IW{1,1}(2,:)'" : Constant  Value=[-0.2427812346794631093160887758131138980388641357421875;-0.3975073394410186811143148588598705828189849853515625;0.846759284206487716772926432895474135875701904296875]
      mask Display: e = 0.06;c1 = [120 150 230]/255;c2 = ([120 150 230]+0)/383;c3 = ([120 150 230]+128)/383;patch([0 1 1 0],[0 0 1 1],c1);patch([0 1 1 1-e 1-e 0+e],[0 0 1 1-e 0+e 0+e],c2);patch([0 0 1 1-e 0+e 0+e],[0 1 1 1-e 1-e 0+e],c3);plot([0 1 1 0 0],[0 0 1 1 0]);disp('Weights');
  "IW{1,1}(3,:)'" : Constant  Value=[0.6342072601445176704970663195126689970493316650390625;-0.00895304815988059825293543525503991986624896526336669921875;-0.224184690646384188195128217557794414460659027099609375]
      mask Display: e = 0.06;c1 = [120 150 230]/255;c2 = ([120 150 230]+0)/383;c3 = ([120 150 230]+128)/383;patch([0 1 1 0],[0 0 1 1],c1);patch([0 1 1 1-e 1-e 0+e],[0 0 1 1-e 0+e 0+e],c2);patch([0 0 1 1-e 0+e 0+e],[0 1 1 1-e 1-e 0+e],c3);plot([0 1 1 0 0],[0 0 1 1 0]);disp('Weights');
  "IW{1,1}(4,:)'" : Constant  Value=[0.1494721401572099706012153319534263573586940765380859375;-3.79655727337768933438155727344565093517303466796875;-0.259951840846281923003147085182718001306056976318359375]
      mask Display: e = 0.06;c1 = [120 150 230]/255;c2 = ([120 150 230]+0)/383;c3 = ([120 150 230]+128)/383;patch([0 1 1 0],[0 0 1 1],c1);patch([0 1 1 1-e 1-e 0+e],[0 0 1 1-e 0+e 0+e],c2);patch([0 0 1 1-e 0+e 0+e],[0 1 1 1-e 1-e 0+e],c3);plot([0 1 1 0 0],[0 0 1 1 0]);disp('Weights');
  "IW{1,1}(5,:)'" : Constant  Value=[-0.394891528062779328944742474050144664943218231201171875;0.47694583369787924009841617589700035750865936279296875;0.73099358430844196821141167674795724451541900634765625]
      mask Display: e = 0.06;c1 = [120 150 230]/255;c2 = ([120 150 230]+0)/383;c3 = ([120 150 230]+128)/383;patch([0 1 1 0],[0 0 1 1],c1);patch([0 1 1 1-e 1-e 0+e],[0 0 1 1-e 0+e 0+e],c2);patch([0 0 1 1-e 0+e 0+e],[0 1 1 1-e 1-e 0+e],c3);plot([0 1 1 0 0],[0 0 1 1 0]);disp('Weights');
  "IW{1,1}(6,:)'" : Constant  Value=[0.8198611307322225538740667616366408765316009521484375;-0.27657710858366491013526911046938039362430572509765625;0.0925979125423994908761216038328711874783039093017578125]
      mask Display: e = 0.06;c1 = [120 150 230]/255;c2 = ([120 150 230]+0)/383;c3 = ([120 150 230]+128)/383;patch([0 1 1 0],[0 0 1 1],c1);patch([0 1 1 1-e 1-e 0+e],[0 0 1 1-e 0+e 0+e],c2);patch([0 0 1 1-e 0+e 0+e],[0 1 1 1-e 1-e 0+e],c3);plot([0 1 1 0 0],[0 0 1 1 0]);disp('Weights');
  "IW{1,1}(7,:)'" : Constant  Value=[0.17244192330773289167922257547616027295589447021484375;1.8056025840962630635289087877026759088039398193359375;0.07073872111181446487027102421052404679358005523681640625]
      mask Display: e = 0.06;c1 = [120 150 230]/255;c2 = ([120 150 230]+0)/383;c3 = ([120 150 230]+128)/383;patch([0 1 1 0],[0 0 1 1],c1);patch([0 1 1 1-e 1-e 0+e],[0 0 1 1-e 0+e 0+e],c2);patch([0 0 1 1-e 0+e 0+e],[0 1 1 1-e 1-e 0+e],c3);plot([0 1 1 0 0],[0 0 1 1 0]);disp('Weights');
  "IW{1,1}(8,:)'" : Constant  Value=[0.100312685796844380803349849884398281574249267578125;-0.658583905704282823734274643356911838054656982421875;-0.7777615531188024622366583571420051157474517822265625]
      mask Display: e = 0.06;c1 = [120 150 230]/255;c2 = ([120 150 230]+0)/383;c3 = ([120 150 230]+128)/383;patch([0 1 1 0],[0 0 1 1],c1);patch([0 1 1 1-e 1-e 0+e],[0 0 1 1-e 0+e 0+e],c2);patch([0 0 1 1-e 0+e 0+e],[0 1 1 1-e 1-e 0+e],c3);plot([0 1 1 0 0],[0 0 1 1 0]);disp('Weights');
  "IW{1,1}(9,:)'" : Constant  Value=[0.225531698608438191389069515935261733829975128173828125;-0.54762037183419420838248470317921601235866546630859375;-0.485090201703608669969725042392383329570293426513671875]
      mask Display: e = 0.06;c1 = [120 150 230]/255;c2 = ([120 150 230]+0)/383;c3 = ([120 150 230]+128)/383;patch([0 1 1 0],[0 0 1 1],c1);patch([0 1 1 1-e 1-e 0+e],[0 0 1 1-e 0+e 0+e],c2);patch([0 0 1 1-e 0+e 0+e],[0 1 1 1-e 1-e 0+e],c3);plot([0 1 1 0 0],[0 0 1 1 0]);disp('Weights');
  Mux : Mux  Inputs=10
      mask Display: e = 0.06;c1 = [120 150 230]/255;c2 = ([120 150 230]+0)/383;c3 = ([120 150 230]+128)/383;patch([0 1 1 0],[0 0 1 1],c1);patch([0 1 1 1-e 1-e 0+e],[0 0 1 1-e 0+e 0+e],c2);patch([0 0 1 1-e 0+e 0+e],[0 1 1 1-e 1-e 0+e],c3);plot([0 1 1 0 0],[0 0 1 1 0]);disp('Mux');
  dotprod{1..10} (10 alike) : neural/Weight Functions/dotprod
  "iz{1,1}" : Outport
      mask Display: e = 0.06;c1 = [120 230 180]/255;c2 = ([120 230 180]+0)/(256+128);c3 = ([120 230 180]+128)/(256+128);patch([0 1 1 0],[0 0 1 1],c1);patch([0 1 1 1-e 1-e 0+e],[0 0 1 1-e 0+e 0+e],c2);patch([0 0 1 1-e 0+e 0+e],[0 1 1 1-e 1-e 0+e],c3);plot([0 1 1 0 0],[0 0 1 1 0]);
  wires:
  "IW{1,1}(1,:)'"/1 -> dotprod1/1
  "pd{1,1}"/1 -> dotprod1/2, dotprod2/2, dotprod3/2, dotprod4/2, dotprod5/2, dotprod6/2, dotprod7/2, dotprod8/2, dotprod9/2, dotprod10/2
  dotprod1/1 -> Mux/1
  "IW{1,1}(2,:)'"/1 -> dotprod2/1
  dotprod2/1 -> Mux/2
  "IW{1,1}(3,:)'"/1 -> dotprod3/1
  dotprod3/1 -> Mux/3
  "IW{1,1}(4,:)'"/1 -> dotprod4/1
  dotprod4/1 -> Mux/4
  "IW{1,1}(5,:)'"/1 -> dotprod5/1
  dotprod5/1 -> Mux/5
  "IW{1,1}(6,:)'"/1 -> dotprod6/1
  dotprod6/1 -> Mux/6
  "IW{1,1}(7,:)'"/1 -> dotprod7/1
  dotprod7/1 -> Mux/7
  "IW{1,1}(8,:)'"/1 -> dotprod8/1
  dotprod8/1 -> Mux/8
  "IW{1,1}(9,:)'"/1 -> dotprod9/1
  dotprod9/1 -> Mux/9
  "IW{1,1}(10,:)'"/1 -> dotprod10/1
  dotprod10/1 -> Mux/10
  Mux/1 -> "iz{1,1}"/1

== system ACC_FFNN_trainlm_10_10_10_Nor_Sat_Feb_15_RepFast/Feed-Forward Neural Network/Layer 2/Delays 1 ==
  "p{2}" : Inport  PortDimensions=10
      mask Display: e = 0.06;c1 = [120 230 180]/255;c2 = ([120 230 180]+0)/(256+128);c3 = ([120 230 180]+128)/(256+128);patch([0 1 1 0],[0 0 1 1],c1);patch([0 1 1 1-e 1-e 0+e],[0 0 1 1-e 0+e 0+e],c2);patch([0 0 1 1-e 0+e 0+e],[0 1 1 1-e 1-e 0+e],c3);plot([0 1 1 0 0],[0 0 1 1 0]);
  mux : Mux  Inputs=1
      mask Display: e = 0.06;c1 = [120 150 230]/255;c2 = ([120 150 230]+0)/383;c3 = ([120 150 230]+128)/383;patch([0 1 1 0],[0 0 1 1],c1);patch([0 1 1 1-e 1-e 0+e],[0 0 1 1-e 0+e 0+e],c2);patch([0 0 1 1-e 0+e 0+e],[0 1 1 1-e 1-e 0+e],c3);plot([0 1 1 0 0],[0 0 1 1 0]);disp('Mux')
  "pd{2,1}" : Outport
      mask Display: e = 0.06;c1 = [120 230 180]/255;c2 = ([120 230 180]+0)/(256+128);c3 = ([120 230 180]+128)/(256+128);patch([0 1 1 0],[0 0 1 1],c1);patch([0 1 1 1-e 1-e 0+e],[0 0 1 1-e 0+e 0+e],c2);patch([0 0 1 1-e 0+e 0+e],[0 1 1 1-e 1-e 0+e],c3);plot([0 1 1 0 0],[0 0 1 1 0]);
  wires:
  "p{2}"/1 -> mux/1
  mux/1 -> "pd{2,1}"/1

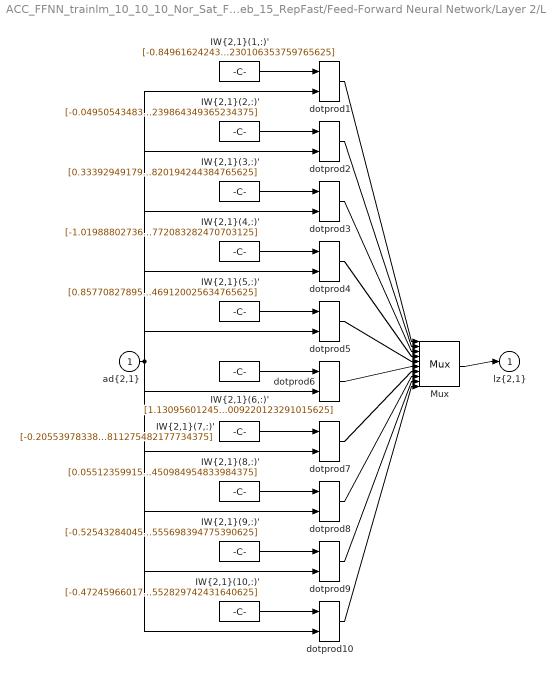
== system ACC_FFNN_trainlm_10_10_10_Nor_Sat_Feb_15_RepFast/Feed-Forward Neural Network/Layer 2/LW{2,1} ==
  "ad{2,1}" : Inport  PortDimensions=10
      mask Display: e = 0.06;c1 = [120 230 180]/255;c2 = ([120 230 180]+0)/(256+128);c3 = ([120 230 180]+128)/(256+128);patch([0 1 1 0],[0 0 1 1],c1);patch([0 1 1 1-e 1-e 0+e],[0 0 1 1-e 0+e 0+e],c2);patch([0 0 1 1-e 0+e 0+e],[0 1 1 1-e 1-e 0+e],c3);plot([0 1 1 0 0],[0 0 1 1 0]);
  "IW{2,1}(1,:)'" : Constant  Value=[-0.8496162424327458051465100652421824634075164794921875;0.9261770785738259181840703604393638670444488525390625;-0.99276634292566467987484202240011654794216156005859375;-0.854124479033524952598099844180978834629058837890625;-0.939430649497594583152704217354767024517059326171875;-0.64922704256248930931860741111449897289276123046875;-0.88176183921681994259955672532669268548488616943359375;0.31921050581661436496005990193225443363189697265625;-0.6532227737619888952025348771712742745876312255859375;-0.416913192959735445786151331049040891230106353759765625]
      mask Display: e = 0.06;c1 = [120 150 230]/255;c2 = ([120 150 230]+0)/383;c3 = ([120 150 230]+128)/383;patch([0 1 1 0],[0 0 1 1],c1);patch([0 1 1 1-e 1-e 0+e],[0 0 1 1-e 0+e 0+e],c2);patch([0 0 1 1-e 0+e 0+e],[0 1 1 1-e 1-e 0+e],c3);plot([0 1 1 0 0],[0 0 1 1 0]);disp('weights');
  "IW{2,1}(10,:)'" : Constant  Value=[-0.472459660174641749019741610027267597615718841552734375;0.9759640063232655204927823433536104857921600341796875;0.2242069978064993307498298236168920993804931640625;-1.883629447495826614300540313706733286380767822265625;0.2263507471964857631352430189508595503866672515869140625;0.265375718038904528928156878464506007730960845947265625;-0.68665609448952891202822002014727331697940826416015625;-0.733657984785676564598588811350055038928985595703125;0.256032053797389635985126687955926172435283660888671875;-0.108171770774200981524160170010873116552829742431640625]
      mask Display: e = 0.06;c1 = [120 150 230]/255;c2 = ([120 150 230]+0)/383;c3 = ([120 150 230]+128)/383;patch([0 1 1 0],[0 0 1 1],c1);patch([0 1 1 1-e 1-e 0+e],[0 0 1 1-e 0+e 0+e],c2);patch([0 0 1 1-e 0+e 0+e],[0 1 1 1-e 1-e 0+e],c3);plot([0 1 1 0 0],[0 0 1 1 0]);disp('weights');
  "IW{2,1}(2,:)'" : Constant  Value=[-0.049505434830052597039440342996385879814624786376953125;0.0936114374779359881273421706282533705234527587890625;0.79088401944895625472753408757853321731090545654296875;0.89997727349861833534561128544737584888935089111328125;0.339012979365227951067396361395367421209812164306640625;-0.5313179840368149609020065327058546245098114013671875;-0.08671245200100409500354459169102483429014682769775390625;0.0371898850210763409762648734613321721553802490234375;-0.2181128966970412863535244696322479285299777984619140625;-1.828083911924957671857328023179434239864349365234375]
      mask Display: e = 0.06;c1 = [120 150 230]/255;c2 = ([120 150 230]+0)/383;c3 = ([120 150 230]+128)/383;patch([0 1 1 0],[0 0 1 1],c1);patch([0 1 1 1-e 1-e 0+e],[0 0 1 1-e 0+e 0+e],c2);patch([0 0 1 1-e 0+e 0+e],[0 1 1 1-e 1-e 0+e],c3);plot([0 1 1 0 0],[0 0 1 1 0]);disp('weights');
  "IW{2,1}(3,:)'" : Constant  Value=[0.3339294917908011139928703414625488221645355224609375;0.042271661608002997212452100939117372035980224609375;0.77423239971629931321928097531781531870365142822265625;-0.4416060312519818342735788974096067249774932861328125;0.070799191167918607003883835204760544002056121826171875;-0.5232302809542692667577057363814674317836761474609375;1.0787096841189203200173096774960868060588836669921875;0.9459491095277250405359836804564110934734344482421875;0.6627594856781391374767054003314115107059478759765625;-3.350297647252054478173022289411164820194244384765625]
      mask Display: e = 0.06;c1 = [120 150 230]/255;c2 = ([120 150 230]+0)/383;c3 = ([120 150 230]+128)/383;patch([0 1 1 0],[0 0 1 1],c1);patch([0 1 1 1-e 1-e 0+e],[0 0 1 1-e 0+e 0+e],c2);patch([0 0 1 1-e 0+e 0+e],[0 1 1 1-e 1-e 0+e],c3);plot([0 1 1 0 0],[0 0 1 1 0]);disp('weights');
  "IW{2,1}(4,:)'" : Constant  Value=[-1.019888027360702498214095612638629972934722900390625;-0.5368112265829523277460566532681696116924285888671875;1.041629176342071527727739521651528775691986083984375;0.462449844300148849018938790322863496840000152587890625;0.084107056986276018673009957637987099587917327880859375;-0.72207555126079825402740652862121351063251495361328125;-0.322765431292603988122635882973554544150829315185546875;0.297982985424712243371914155432023108005523681640625;0.6066325855726779625598510392592288553714752197265625;2.330883155311792354069666544091887772083282470703125]
      mask Display: e = 0.06;c1 = [120 150 230]/255;c2 = ([120 150 230]+0)/383;c3 = ([120 150 230]+128)/383;patch([0 1 1 0],[0 0 1 1],c1);patch([0 1 1 1-e 1-e 0+e],[0 0 1 1-e 0+e 0+e],c2);patch([0 0 1 1-e 0+e 0+e],[0 1 1 1-e 1-e 0+e],c3);plot([0 1 1 0 0],[0 0 1 1 0]);disp('weights');
  "IW{2,1}(5,:)'" : Constant  Value=[0.8577082789560892539526548716821707785129547119140625;-0.0222045121596661232388214557431638240814208984375;-0.802575442688851392603055501240305602550506591796875;0.43007415680138816327371387160383164882659912109375;0.809444476134725476867970428429543972015380859375;-0.0201972229755522647565157967619597911834716796875;0.04329968492856739459284654003567993640899658203125;0.60066115070480297077892828383482992649078369140625;-0.8790576416602127185484505389467813074588775634765625;-0.665663180170688040249160621897317469120025634765625]
      mask Display: e = 0.06;c1 = [120 150 230]/255;c2 = ([120 150 230]+0)/383;c3 = ([120 150 230]+128)/383;patch([0 1 1 0],[0 0 1 1],c1);patch([0 1 1 1-e 1-e 0+e],[0 0 1 1-e 0+e 0+e],c2);patch([0 0 1 1-e 0+e 0+e],[0 1 1 1-e 1-e 0+e],c3);plot([0 1 1 0 0],[0 0 1 1 0]);disp('weights');
  "IW{2,1}(6,:)'" : Constant  Value=[1.1309560124591644392211264857905916869640350341796875;0.248120176347379040038276798441074788570404052734375;-0.0628173500868061396307240329406340606510639190673828125;1.55512406309582384977829860872589051723480224609375;0.2197332968451168877521695321775041520595550537109375;0.01274078071968580590234143556926937890239059925079345703125;-1.6896147136380832431967746742884628474712371826171875;-0.0924045825461610181861260571167804300785064697265625;-0.2015579014878563501866892693215049803256988525390625;-1.6577258977847348919709702386171557009220123291015625]
      mask Display: e = 0.06;c1 = [120 150 230]/255;c2 = ([120 150 230]+0)/383;c3 = ([120 150 230]+128)/383;patch([0 1 1 0],[0 0 1 1],c1);patch([0 1 1 1-e 1-e 0+e],[0 0 1 1-e 0+e 0+e],c2);patch([0 0 1 1-e 0+e 0+e],[0 1 1 1-e 1-e 0+e],c3);plot([0 1 1 0 0],[0 0 1 1 0]);disp('weights');
  "IW{2,1}(7,:)'" : Constant  Value=[-0.2055397833860117540183409801102243363857269287109375;0.3582710817314953555268175477976910769939422607421875;0.45143170587027003914926126526552252471446990966796875;2.487530611421458814902507583610713481903076171875;0.25444374894181909230184146508690901100635528564453125;0.71002023217130394439067231360240839421749114990234375;0.0754730933538476922439741656489786691963672637939453125;-0.1352169924330766104247913972358219325542449951171875;0.0537293483998199927764716221645358018577098846435546875;-0.1608744893919090424017070972695364616811275482177734375]
      mask Display: e = 0.06;c1 = [120 150 230]/255;c2 = ([120 150 230]+0)/383;c3 = ([120 150 230]+128)/383;patch([0 1 1 0],[0 0 1 1],c1);patch([0 1 1 1-e 1-e 0+e],[0 0 1 1-e 0+e 0+e],c2);patch([0 0 1 1-e 0+e 0+e],[0 1 1 1-e 1-e 0+e],c3);plot([0 1 1 0 0],[0 0 1 1 0]);disp('weights');
  "IW{2,1}(8,:)'" : Constant  Value=[0.05512359915568987300815706475987099111080169677734375;-0.208969568662813909298847647733055055141448974609375;0.2352851189098039974556542119898949749767780303955078125;-1.550100254859075210589480775524862110614776611328125;0.6286560408082408901719873028923757374286651611328125;0.350651326424857467944917743807309307157993316650390625;1.0521665278259317855003018848947249352931976318359375;0.6506275908040912714369596869801171123981475830078125;-0.1662692996840871295649577632502769120037555694580078125;-0.8298127683754985550734772914438508450984954833984375]
      mask Display: e = 0.06;c1 = [120 150 230]/255;c2 = ([120 150 230]+0)/383;c3 = ([120 150 230]+128)/383;patch([0 1 1 0],[0 0 1 1],c1);patch([0 1 1 1-e 1-e 0+e],[0 0 1 1-e 0+e 0+e],c2);patch([0 0 1 1-e 0+e 0+e],[0 1 1 1-e 1-e 0+e],c3);plot([0 1 1 0 0],[0 0 1 1 0]);disp('weights');
  "IW{2,1}(9,:)'" : Constant  Value=[-0.5254328404569570398763289631460793316364288330078125;-0.2651267029110468964603342101327143609523773193359375;-0.726893725289260661526213880279101431369781494140625;0.3974916646695889621554442783235572278499603271484375;0.6109788490593712761977940317592583596706390380859375;0.00094324830968606221404115785844624042510986328125;0.4448791847336845961535800597630441188812255859375;-0.8330603702821719469540084901382215321063995361328125;0.3137197819474144555584871341125108301639556884765625;-0.0206247239679522298416713965707458555698394775390625]
      mask Display: e = 0.06;c1 = [120 150 230]/255;c2 = ([120 150 230]+0)/383;c3 = ([120 150 230]+128)/383;patch([0 1 1 0],[0 0 1 1],c1);patch([0 1 1 1-e 1-e 0+e],[0 0 1 1-e 0+e 0+e],c2);patch([0 0 1 1-e 0+e 0+e],[0 1 1 1-e 1-e 0+e],c3);plot([0 1 1 0 0],[0 0 1 1 0]);disp('weights');
  Mux : Mux  Inputs=10
      mask Display: e = 0.06;c1 = [120 150 230]/255;c2 = ([120 150 230]+0)/383;c3 = ([120 150 230]+128)/383;patch([0 1 1 0],[0 0 1 1],c1);patch([0 1 1 1-e 1-e 0+e],[0 0 1 1-e 0+e 0+e],c2);patch([0 0 1 1-e 0+e 0+e],[0 1 1 1-e 1-e 0+e],c3);plot([0 1 1 0 0],[0 0 1 1 0]);disp('Mux');
  dotprod{1..10} (10 alike) : neural/Weight Functions/dotprod
  "lz{2,1}" : Outport
      mask Display: e = 0.06;c1 = [120 230 180]/255;c2 = ([120 230 180]+0)/(256+128);c3 = ([120 230 180]+128)/(256+128);patch([0 1 1 0],[0 0 1 1],c1);patch([0 1 1 1-e 1-e 0+e],[0 0 1 1-e 0+e 0+e],c2);patch([0 0 1 1-e 0+e 0+e],[0 1 1 1-e 1-e 0+e],c3);plot([0 1 1 0 0],[0 0 1 1 0]);
  wires:
  "IW{2,1}(1,:)'"/1 -> dotprod1/1
  "ad{2,1}"/1 -> dotprod1/2, dotprod2/2, dotprod3/2, dotprod4/2, dotprod5/2, dotprod6/2, dotprod7/2, dotprod8/2, dotprod9/2, dotprod10/2
  dotprod1/1 -> Mux/1
  "IW{2,1}(2,:)'"/1 -> dotprod2/1
  dotprod2/1 -> Mux/2
  "IW{2,1}(3,:)'"/1 -> dotprod3/1
  dotprod3/1 -> Mux/3
  "IW{2,1}(4,:)'"/1 -> dotprod4/1
  dotprod4/1 -> Mux/4
  "IW{2,1}(5,:)'"/1 -> dotprod5/1
  dotprod5/1 -> Mux/5
  "IW{2,1}(6,:)'"/1 -> dotprod6/1
  dotprod6/1 -> Mux/6
  "IW{2,1}(7,:)'"/1 -> dotprod7/1
  dotprod7/1 -> Mux/7
  "IW{2,1}(8,:)'"/1 -> dotprod8/1
  dotprod8/1 -> Mux/8
  "IW{2,1}(9,:)'"/1 -> dotprod9/1
  dotprod9/1 -> Mux/9
  "IW{2,1}(10,:)'"/1 -> dotprod10/1
  dotprod10/1 -> Mux/10
  Mux/1 -> "lz{2,1}"/1

== system ACC_FFNN_trainlm_10_10_10_Nor_Sat_Feb_15_RepFast/Feed-Forward Neural Network/Layer 3/Delays 1 ==
  "p{3}" : Inport  PortDimensions=10
      mask Display: e = 0.06;c1 = [120 230 180]/255;c2 = ([120 230 180]+0)/(256+128);c3 = ([120 230 180]+128)/(256+128);patch([0 1 1 0],[0 0 1 1],c1);patch([0 1 1 1-e 1-e 0+e],[0 0 1 1-e 0+e 0+e],c2);patch([0 0 1 1-e 0+e 0+e],[0 1 1 1-e 1-e 0+e],c3);plot([0 1 1 0 0],[0 0 1 1 0]);
  mux : Mux  Inputs=1
      mask Display: e = 0.06;c1 = [120 150 230]/255;c2 = ([120 150 230]+0)/383;c3 = ([120 150 230]+128)/383;patch([0 1 1 0],[0 0 1 1],c1);patch([0 1 1 1-e 1-e 0+e],[0 0 1 1-e 0+e 0+e],c2);patch([0 0 1 1-e 0+e 0+e],[0 1 1 1-e 1-e 0+e],c3);plot([0 1 1 0 0],[0 0 1 1 0]);disp('Mux')
  "pd{3,2}" : Outport
      mask Display: e = 0.06;c1 = [120 230 180]/255;c2 = ([120 230 180]+0)/(256+128);c3 = ([120 230 180]+128)/(256+128);patch([0 1 1 0],[0 0 1 1],c1);patch([0 1 1 1-e 1-e 0+e],[0 0 1 1-e 0+e 0+e],c2);patch([0 0 1 1-e 0+e 0+e],[0 1 1 1-e 1-e 0+e],c3);plot([0 1 1 0 0],[0 0 1 1 0]);
  wires:
  "p{3}"/1 -> mux/1
  mux/1 -> "pd{3,2}"/1
